simulink model "BCwithBPfix1"  (Simulink 7.0)
settings: Solver=FixedStepDiscrete  StartTime=0.0  StopTime=inf  FixedStep=0.001  RelTol=1e-3
libraries: dspsigops x84, dsPICdrivers x4
settings Model: Creator=Casparus  LastModifiedBy=Casparus  BufferReuse=off
settings OptimizationCC: BlockReduction=off  ConditionallyExecuteInputs=off  InlineParams=on  InlineInvariantSignals=on  OptimizeBlockIOStorage=off  BufferReuse=off  ExpressionFolding=off  LocalBlockOutputs=off  ZeroInternalMemoryAtStartup=off  InitFltsAndDblsToZero=off  EfficientFloat2IntCast=on  OptimizeModelRefInitCode=on
settings DebuggingCC: SignalInfNanChecking=error  ReadBeforeWriteMsg=EnableAllAsError  WriteAfterWriteMsg=EnableAllAsError  WriteAfterReadMsg=EnableAllAsError  AlgebraicLoopMsg=error  ArtificialAlgebraicLoopMsg=error  CheckExecutionContextPreStartOutputMsg=on  CheckExecutionContextRuntimeOutputMsg=on  BlockPriorityViolationMsg=error  SolverPrmCheckMsg=error  InheritedTsInSrcMsg=error  DiscreteInheritContinuousMsg=error  SigSpecEnsureSampleTimeMsg=error  CheckMatrixSingularityMsg=error  IntegerOverflowMsg=error  ParameterUnderflowMsg=error  ParameterPrecisionLossMsg=error  ParameterTunabilityLossMsg=error  UnderSpecifiedDataTypeMsg=error  UnnecessaryDatatypeConvMsg=warning  VectorMatrixConversionMsg=error  FcnCallInpInsideContextMsg=Enable All  SignalLabelMismatchMsg=error  UnconnectedInputMsg=error  UnconnectedOutputMsg=error  UnconnectedLineMsg=error  SFcnCompatibilityMsg=error  BusObjectLabelMismatch=error  RootOutportRequireBusObject=error  AssertControl=DisableAll  ModelReferenceIOMsg=error  ModelReferenceIOMismatchMessage=error  ModelReferenceCSMismatchMessage=warning  UnknownTsInhSupMsg=error  ModelReferenceDataLoggingMessage=error  StrictBusMsg=ErrorLevel1
settings HardwareCC: ProdBitPerInt=16  ProdEndianess=LittleEndian  ProdWordSize=16  ProdHWDeviceType=16-bit Generic
settings RTWCC: SystemTargetFile=dspic.tlc  TemplateMakefile=dspic_pic30_gcc.tmf  PostCodeGenCommand=dsPIC_Compile()  Description=Embedded Target for Microchip dsPIC (real-time)  ProcessScript=dspic_make_rtw_hook
settings CodeAppCC: ForceParamTrailComments=on  IgnoreCustomStorageClasses=off  MangleLength=4  ReqsInCode=on
settings STFCustomTargetCC: GenFloatMathFcnCalls=ANSI_C  ModelReferenceCompliant=off  IncludeMdlTerminateFcn=off  CombineOutputUpdateFcns=on  SuppressErrorStatus=on  ERTCustomFileBanners=on  SupportAbsoluteTime=off  SupportNonFinite=off  SupportContinuousTime=off  SupportNonInlinedSFcns=off  ParenthesesLevel=Maximum  SystemTargetFile=dspic.tlc
settings ERTTargetCC: GenFloatMathFcnCalls=ANSI_C  ModelReferenceCompliant=off  CompOptLevelCompliant=off  IncludeMdlTerminateFcn=off  SuppressErrorStatus=on  SupportAbsoluteTime=off  SupportNonFinite=off  ParenthesesLevel=Maximum  ModelStepFunctionPrototypeControlCompliant=off  ExtModeMexFile=noextcomm  InlinedParameterPlacement=NonHierarchical  ERTSrcFileBannerTemplate=dsPIC_code_template.cgt  ERTHdrFileBannerTemplate=dsPIC_code_template.cgt  ERTDataSrcFileTemplate=dsPIC_code_template.cgt  ERTDataHdrFileTemplate=dsPIC_code_template.cgt  ERTCustomFileTemplate=dsPIC_main.tlc  PreserveExpressionOrder=on  PreserveIfCondition=on
settings CustomProperty: DataType=string  Value=C:\PROGRA~1\MATLAB\R2007b\bin\win32\gmake

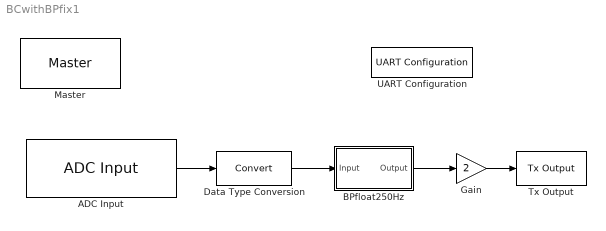
== system BCwithBPfix1 ==
  ADC Input : dsPICdrivers/Peripheral I//O/ADC Input  Tag=dsPIC_ADC  Priority=5  ADC_TYPE=12 bits  ADC_MODE=Continuous Sampling get output vector  NbrSampleStep=1  VoltRefpopup="External Vref+  -  AVss"  OutFormatBitspopup=0000 dddd dddd dddd : Integer  InterruptPriority=6  ANCHANNELS=[0]  MaxName=ANmax = 4096  Rin=1e2  ADCS=3  SAMC=1  Temperature=25  DMAChannel=0  SampleTime=0.001  Status="OK  |  Tsmp=8.000e-007 |  T/Channel=1.200e-005 |  Tall=1.200e-005"
  BPfloat250Hz : Subsystem  Tag=FilterWizardSubSystem
      settings: ErrorFcn=dspFilterRealizedInBasicElemsAlgLoopErrFcnCallback
  Data Type Conversion : DataTypeConversion  OutDataTypeMode=Specify via dialog
  Gain : Gain  Gain=2  ParameterDataType=sfix(16)  ParameterScaling=2^0  OutDataTypeMode=uint8  OutDataType=sfix(16)  OutScaling=2^0
  Master : dsPICdrivers/Master  Tag=dsPIC_MASTER  Priority=1  TimeStepType=Timer1  picType=30f4013  fcy=2.5e6  Quartz_33f=5e6  PLLActive_33f=off  fcyDesired_33f=0  tmr1="[1  2499  0]"  tmr1Info="Time Step : 0.001  ;   Error : 0%  PR1=2499"  tmr2345="[0  0  0  0]"  tmr2345cfg=[-1 -1 -1 -1]  IOautoConf=on  typePort="[ 0  0  0  0  0  0  0  0  0  0  0  0  0  0  0  0  8  0  0  0  0  0  0  0  0  0  0  0  0  0  0  0  0  0  0  0  0  0  0  0  0  0  0  0  0  0  0  0  0  0  0  0  0  0  0  0  0  0  0  0  0  0  0  0  0  0  0  0  0  0  0  0  0  0  0  0  0  0  0  0  0  0  4  5  0  0  0  0  0  0  0  0  0  0  0  0  0  0  0  0  0  0  0  0  0  0  0  0  0  0  0  0 ]"  TRIS="[ 65535  65535  65535  65535  65535  65535  65535 ]"  ADPCFG=0  MasterBusyPort=None  MasterOverloadPort=None  FOSC=XTL  TempProtection_33f=TEMP_ON  FPBOR=PBOR_OFF  PWRT=PWRT_OFF  MCLR=MCLR_DIS  PowerSave=off
  Tx Output : dsPICdrivers/Serial PORT/Tx Output  Tag=dsPIC_TX  Priority=5  UART=1  OrderingInOutPopup=None
  UART Configuration : dsPICdrivers/Serial PORT/UART Configuration  Tag=dsPIC_config_UART  Priority=2  UART=1  proposed_BAUD=9600  ALT_TX_RX=off  InterruptTxWhen=When Transmit Buffer is empty  TXInterruptPri=1  TxBufferSize=32  TXEN=on  InterruptRxWhen=When Receive Buffer is full (contain 4 characters)  RXInterruptPri=1  RxBufferSize=32  BAUD=9600  UxBRG=15  Info="UxBRG = 15   ||  Real Baud : 9766   ||  % error : 1.7253  ||  max 0.97656 Bytes / Step"  RealBaud=0
  wires:
  Gain/1 -> Tx Output/1
  ADC Input/1 -> Data Type Conversion/1
  Data Type Conversion/1 -> BPfloat250Hz/1(Input)
  BPfloat250Hz/1(Output) -> Gain/1

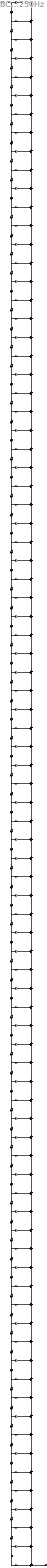
== system BCwithBPfix1/BPfloat250Hz ==
  Input : Inport
  BodyDelay{2..85} (84 alike) : dspsigops/Delay  Orientation=down  dly_unit=Samples  delay=1  ic_detail=off  dif_ic_for_ch=off  dif_ic_for_dly=off  ic=0  reset_popup=None
  BodyLSum{2..84} (83 alike) : Sum  Orientation=down  Inputs=++|  OutScaling=1  RndMeth=Nearest  SaturateOnIntegerOverflow=on
  BodyLSum85 : Sum  Inputs=++|  OutScaling=1  RndMeth=Nearest  SaturateOnIntegerOverflow=on
  b(1) : Gain  Gain=-0.00011400410035938231  ParameterDataTypeMode=Specify via dialog  ParameterDataType=float('double')  ParameterScalingMode=Use specified scaling  ParameterScaling=1  OutScaling=1  RndMeth=Nearest  SaturateOnIntegerOverflow=on
  b(10) : Gain  Gain=0.00076528749014445803  ParameterDataTypeMode=Specify via dialog  ParameterDataType=float('double')  ParameterScalingMode=Use specified scaling  ParameterScaling=1  OutScaling=1  RndMeth=Nearest  SaturateOnIntegerOverflow=on
  b(11) : Gain  Gain=-0.00055653560863696205  ParameterDataTypeMode=Specify via dialog  ParameterDataType=float('double')  ParameterScalingMode=Use specified scaling  ParameterScaling=1  OutScaling=1  RndMeth=Nearest  SaturateOnIntegerOverflow=on
  b(12) : Gain  Gain=-0.0017653960169033756  ParameterDataTypeMode=Specify via dialog  ParameterDataType=float('double')  ParameterScalingMode=Use specified scaling  ParameterScaling=1  OutScaling=1  RndMeth=Nearest  SaturateOnIntegerOverflow=on
  b(13) : Gain  Gain=0.00080126316068455581  ParameterDataTypeMode=Specify via dialog  ParameterDataType=float('double')  ParameterScalingMode=Use specified scaling  ParameterScaling=1  OutScaling=1  RndMeth=Nearest  SaturateOnIntegerOverflow=on
  b(14) : Gain  Gain=0.0033745175704345386  ParameterDataTypeMode=Specify via dialog  ParameterDataType=float('double')  ParameterScalingMode=Use specified scaling  ParameterScaling=1  OutScaling=1  RndMeth=Nearest  SaturateOnIntegerOverflow=on
  b(15) : Gain  Gain=-0.00084331270675375408  ParameterDataTypeMode=Specify via dialog  ParameterDataType=float('double')  ParameterScalingMode=Use specified scaling  ParameterScaling=1  OutScaling=1  RndMeth=Nearest  SaturateOnIntegerOverflow=on
  b(16) : Gain  Gain=-0.0057166316791322285  ParameterDataTypeMode=Specify via dialog  ParameterDataType=float('double')  ParameterScalingMode=Use specified scaling  ParameterScaling=1  OutScaling=1  RndMeth=Nearest  SaturateOnIntegerOverflow=on
  b(17) : Gain  Gain=0.0004479504040917559  ParameterDataTypeMode=Specify via dialog  ParameterDataType=float('double')  ParameterScalingMode=Use specified scaling  ParameterScaling=1  OutScaling=1  RndMeth=Nearest  SaturateOnIntegerOverflow=on
  b(18) : Gain  Gain=0.0088411131476842132  ParameterDataTypeMode=Specify via dialog  ParameterDataType=float('double')  ParameterScalingMode=Use specified scaling  ParameterScaling=1  OutScaling=1  RndMeth=Nearest  SaturateOnIntegerOverflow=on
  b(19) : Gain  Gain=0.00067442731314515544  ParameterDataTypeMode=Specify via dialog  ParameterDataType=float('double')  ParameterScalingMode=Use specified scaling  ParameterScaling=1  OutScaling=1  RndMeth=Nearest  SaturateOnIntegerOverflow=on
  b(2) : Gain  Gain=-0.00012559964702687091  ParameterDataTypeMode=Specify via dialog  ParameterDataType=float('double')  ParameterScalingMode=Use specified scaling  ParameterScaling=1  OutScaling=1  RndMeth=Nearest  SaturateOnIntegerOverflow=on
  b(20) : Gain  Gain=-0.012691969772935312  ParameterDataTypeMode=Specify via dialog  ParameterDataType=float('double')  ParameterScalingMode=Use specified scaling  ParameterScaling=1  OutScaling=1  RndMeth=Nearest  SaturateOnIntegerOverflow=on
  b(21) : Gain  Gain=-0.0028302241701637521  ParameterDataTypeMode=Specify via dialog  ParameterDataType=float('double')  ParameterScalingMode=Use specified scaling  ParameterScaling=1  OutScaling=1  RndMeth=Nearest  SaturateOnIntegerOverflow=on
  b(22) : Gain  Gain=0.017080765259904356  ParameterDataTypeMode=Specify via dialog  ParameterDataType=float('double')  ParameterScalingMode=Use specified scaling  ParameterScaling=1  OutScaling=1  RndMeth=Nearest  SaturateOnIntegerOverflow=on
  b(23) : Gain  Gain=0.0062943956875770521  ParameterDataTypeMode=Specify via dialog  ParameterDataType=float('double')  ParameterScalingMode=Use specified scaling  ParameterScaling=1  OutScaling=1  RndMeth=Nearest  SaturateOnIntegerOverflow=on
  b(24) : Gain  Gain=-0.021679640249729602  ParameterDataTypeMode=Specify via dialog  ParameterDataType=float('double')  ParameterScalingMode=Use specified scaling  ParameterScaling=1  OutScaling=1  RndMeth=Nearest  SaturateOnIntegerOverflow=on
  b(25) : Gain  Gain=-0.011251464760916772  ParameterDataTypeMode=Specify via dialog  ParameterDataType=float('double')  ParameterScalingMode=Use specified scaling  ParameterScaling=1  OutScaling=1  RndMeth=Nearest  SaturateOnIntegerOverflow=on
  b(26) : Gain  Gain=0.026040044883898328  ParameterDataTypeMode=Specify via dialog  ParameterDataType=float('double')  ParameterScalingMode=Use specified scaling  ParameterScaling=1  OutScaling=1  RndMeth=Nearest  SaturateOnIntegerOverflow=on
  b(27) : Gain  Gain=0.01774070618611993  ParameterDataTypeMode=Specify via dialog  ParameterDataType=float('double')  ParameterScalingMode=Use specified scaling  ParameterScaling=1  OutScaling=1  RndMeth=Nearest  SaturateOnIntegerOverflow=on
  b(28) : Gain  Gain=-0.029634639615999717  ParameterDataTypeMode=Specify via dialog  ParameterDataType=float('double')  ParameterScalingMode=Use specified scaling  ParameterScaling=1  OutScaling=1  RndMeth=Nearest  SaturateOnIntegerOverflow=on
  b(29) : Gain  Gain=-0.025613322377926483  ParameterDataTypeMode=Specify via dialog  ParameterDataType=float('double')  ParameterScalingMode=Use specified scaling  ParameterScaling=1  OutScaling=1  RndMeth=Nearest  SaturateOnIntegerOverflow=on
  b(3) : Gain  Gain=0.00014771328412910959  ParameterDataTypeMode=Specify via dialog  ParameterDataType=float('double')  ParameterScalingMode=Use specified scaling  ParameterScaling=1  OutScaling=1  RndMeth=Nearest  SaturateOnIntegerOverflow=on
  b(30) : Gain  Gain=0.031923272179050548  ParameterDataTypeMode=Specify via dialog  ParameterDataType=float('double')  ParameterScalingMode=Use specified scaling  ParameterScaling=1  OutScaling=1  RndMeth=Nearest  SaturateOnIntegerOverflow=on
  b(31) : Gain  Gain=0.034515179237363247  ParameterDataTypeMode=Specify via dialog  ParameterDataType=float('double')  ParameterScalingMode=Use specified scaling  ParameterScaling=1  OutScaling=1  RndMeth=Nearest  SaturateOnIntegerOverflow=on
  b(32) : Gain  Gain=-0.032431430566267301  ParameterDataTypeMode=Specify via dialog  ParameterDataType=float('double')  ParameterScalingMode=Use specified scaling  ParameterScaling=1  OutScaling=1  RndMeth=Nearest  SaturateOnIntegerOverflow=on
  b(33) : Gain  Gain=-0.043899732573517758  ParameterDataTypeMode=Specify via dialog  ParameterDataType=float('double')  ParameterScalingMode=Use specified scaling  ParameterScaling=1  OutScaling=1  RndMeth=Nearest  SaturateOnIntegerOverflow=on
  b(34) : Gain  Gain=0.030828713556614439  ParameterDataTypeMode=Specify via dialog  ParameterDataType=float('double')  ParameterScalingMode=Use specified scaling  ParameterScaling=1  OutScaling=1  RndMeth=Nearest  SaturateOnIntegerOverflow=on
  b(35) : Gain  Gain=0.053075176357706616  ParameterDataTypeMode=Specify via dialog  ParameterDataType=float('double')  ParameterScalingMode=Use specified scaling  ParameterScaling=1  OutScaling=1  RndMeth=Nearest  SaturateOnIntegerOverflow=on
  b(36) : Gain  Gain=-0.026994527169246309  ParameterDataTypeMode=Specify via dialog  ParameterDataType=float('double')  ParameterScalingMode=Use specified scaling  ParameterScaling=1  OutScaling=1  RndMeth=Nearest  SaturateOnIntegerOverflow=on
  b(37) : Gain  Gain=-0.061279551446267191  ParameterDataTypeMode=Specify via dialog  ParameterDataType=float('double')  ParameterScalingMode=Use specified scaling  ParameterScaling=1  OutScaling=1  RndMeth=Nearest  SaturateOnIntegerOverflow=on
  b(38) : Gain  Gain=0.021056309766186106  ParameterDataTypeMode=Specify via dialog  ParameterDataType=float('double')  ParameterScalingMode=Use specified scaling  ParameterScaling=1  OutScaling=1  RndMeth=Nearest  SaturateOnIntegerOverflow=on
  b(39) : Gain  Gain=0.067775120580984796  ParameterDataTypeMode=Specify via dialog  ParameterDataType=float('double')  ParameterScalingMode=Use specified scaling  ParameterScaling=1  OutScaling=1  RndMeth=Nearest  SaturateOnIntegerOverflow=on
  b(4) : Gain  Gain=5.5446602993773556e-005  ParameterDataTypeMode=Specify via dialog  ParameterDataType=float('double')  ParameterScalingMode=Use specified scaling  ParameterScaling=1  OutScaling=1  RndMeth=Nearest  SaturateOnIntegerOverflow=on
  b(40) : Gain  Gain=-0.013392258720000015  ParameterDataTypeMode=Specify via dialog  ParameterDataType=float('double')  ParameterScalingMode=Use specified scaling  ParameterScaling=1  OutScaling=1  RndMeth=Nearest  SaturateOnIntegerOverflow=on
  b(41) : Gain  Gain=-0.071946166637857939  ParameterDataTypeMode=Specify via dialog  ParameterDataType=float('double')  ParameterScalingMode=Use specified scaling  ParameterScaling=1  OutScaling=1  RndMeth=Nearest  SaturateOnIntegerOverflow=on
  b(42) : Gain  Gain=0.0045956094220973263  ParameterDataTypeMode=Specify via dialog  ParameterDataType=float('double')  ParameterScalingMode=Use specified scaling  ParameterScaling=1  OutScaling=1  RndMeth=Nearest  SaturateOnIntegerOverflow=on
  b(43) : Gain  Gain=0.073384080651335476  ParameterDataTypeMode=Specify via dialog  ParameterDataType=float('double')  ParameterScalingMode=Use specified scaling  ParameterScaling=1  OutScaling=1  RndMeth=Nearest  SaturateOnIntegerOverflow=on
  b(44) : Gain  Gain=0.0045956094220973263  ParameterDataTypeMode=Specify via dialog  ParameterDataType=float('double')  ParameterScalingMode=Use specified scaling  ParameterScaling=1  OutScaling=1  RndMeth=Nearest  SaturateOnIntegerOverflow=on
  b(45) : Gain  Gain=-0.071946166637857939  ParameterDataTypeMode=Specify via dialog  ParameterDataType=float('double')  ParameterScalingMode=Use specified scaling  ParameterScaling=1  OutScaling=1  RndMeth=Nearest  SaturateOnIntegerOverflow=on
  b(46) : Gain  Gain=-0.013392258720000015  ParameterDataTypeMode=Specify via dialog  ParameterDataType=float('double')  ParameterScalingMode=Use specified scaling  ParameterScaling=1  OutScaling=1  RndMeth=Nearest  SaturateOnIntegerOverflow=on
  b(47) : Gain  Gain=0.067775120580984796  ParameterDataTypeMode=Specify via dialog  ParameterDataType=float('double')  ParameterScalingMode=Use specified scaling  ParameterScaling=1  OutScaling=1  RndMeth=Nearest  SaturateOnIntegerOverflow=on
  b(48) : Gain  Gain=0.021056309766186106  ParameterDataTypeMode=Specify via dialog  ParameterDataType=float('double')  ParameterScalingMode=Use specified scaling  ParameterScaling=1  OutScaling=1  RndMeth=Nearest  SaturateOnIntegerOverflow=on
  b(49) : Gain  Gain=-0.061279551446267191  ParameterDataTypeMode=Specify via dialog  ParameterDataType=float('double')  ParameterScalingMode=Use specified scaling  ParameterScaling=1  OutScaling=1  RndMeth=Nearest  SaturateOnIntegerOverflow=on
  b(5) : Gain  Gain=-5.7332663760778328e-005  ParameterDataTypeMode=Specify via dialog  ParameterDataType=float('double')  ParameterScalingMode=Use specified scaling  ParameterScaling=1  OutScaling=1  RndMeth=Nearest  SaturateOnIntegerOverflow=on
  b(50) : Gain  Gain=-0.026994527169246309  ParameterDataTypeMode=Specify via dialog  ParameterDataType=float('double')  ParameterScalingMode=Use specified scaling  ParameterScaling=1  OutScaling=1  RndMeth=Nearest  SaturateOnIntegerOverflow=on
  b(51) : Gain  Gain=0.053075176357706616  ParameterDataTypeMode=Specify via dialog  ParameterDataType=float('double')  ParameterScalingMode=Use specified scaling  ParameterScaling=1  OutScaling=1  RndMeth=Nearest  SaturateOnIntegerOverflow=on
  b(52) : Gain  Gain=0.030828713556614439  ParameterDataTypeMode=Specify via dialog  ParameterDataType=float('double')  ParameterScalingMode=Use specified scaling  ParameterScaling=1  OutScaling=1  RndMeth=Nearest  SaturateOnIntegerOverflow=on
  b(53) : Gain  Gain=-0.043899732573517758  ParameterDataTypeMode=Specify via dialog  ParameterDataType=float('double')  ParameterScalingMode=Use specified scaling  ParameterScaling=1  OutScaling=1  RndMeth=Nearest  SaturateOnIntegerOverflow=on
  b(54) : Gain  Gain=-0.032431430566267301  ParameterDataTypeMode=Specify via dialog  ParameterDataType=float('double')  ParameterScalingMode=Use specified scaling  ParameterScaling=1  OutScaling=1  RndMeth=Nearest  SaturateOnIntegerOverflow=on
  b(55) : Gain  Gain=0.034515179237363247  ParameterDataTypeMode=Specify via dialog  ParameterDataType=float('double')  ParameterScalingMode=Use specified scaling  ParameterScaling=1  OutScaling=1  RndMeth=Nearest  SaturateOnIntegerOverflow=on
  b(56) : Gain  Gain=0.031923272179050548  ParameterDataTypeMode=Specify via dialog  ParameterDataType=float('double')  ParameterScalingMode=Use specified scaling  ParameterScaling=1  OutScaling=1  RndMeth=Nearest  SaturateOnIntegerOverflow=on
  b(57) : Gain  Gain=-0.025613322377926483  ParameterDataTypeMode=Specify via dialog  ParameterDataType=float('double')  ParameterScalingMode=Use specified scaling  ParameterScaling=1  OutScaling=1  RndMeth=Nearest  SaturateOnIntegerOverflow=on
  b(58) : Gain  Gain=-0.029634639615999717  ParameterDataTypeMode=Specify via dialog  ParameterDataType=float('double')  ParameterScalingMode=Use specified scaling  ParameterScaling=1  OutScaling=1  RndMeth=Nearest  SaturateOnIntegerOverflow=on
  b(59) : Gain  Gain=0.01774070618611993  ParameterDataTypeMode=Specify via dialog  ParameterDataType=float('double')  ParameterScalingMode=Use specified scaling  ParameterScaling=1  OutScaling=1  RndMeth=Nearest  SaturateOnIntegerOverflow=on
  b(6) : Gain  Gain=-2.1431167664734075e-005  ParameterDataTypeMode=Specify via dialog  ParameterDataType=float('double')  ParameterScalingMode=Use specified scaling  ParameterScaling=1  OutScaling=1  RndMeth=Nearest  SaturateOnIntegerOverflow=on
  b(60) : Gain  Gain=0.026040044883898328  ParameterDataTypeMode=Specify via dialog  ParameterDataType=float('double')  ParameterScalingMode=Use specified scaling  ParameterScaling=1  OutScaling=1  RndMeth=Nearest  SaturateOnIntegerOverflow=on
  b(61) : Gain  Gain=-0.011251464760916772  ParameterDataTypeMode=Specify via dialog  ParameterDataType=float('double')  ParameterScalingMode=Use specified scaling  ParameterScaling=1  OutScaling=1  RndMeth=Nearest  SaturateOnIntegerOverflow=on
  b(62) : Gain  Gain=-0.021679640249729602  ParameterDataTypeMode=Specify via dialog  ParameterDataType=float('double')  ParameterScalingMode=Use specified scaling  ParameterScaling=1  OutScaling=1  RndMeth=Nearest  SaturateOnIntegerOverflow=on
  b(63) : Gain  Gain=0.0062943956875770521  ParameterDataTypeMode=Specify via dialog  ParameterDataType=float('double')  ParameterScalingMode=Use specified scaling  ParameterScaling=1  OutScaling=1  RndMeth=Nearest  SaturateOnIntegerOverflow=on
  b(64) : Gain  Gain=0.017080765259904356  ParameterDataTypeMode=Specify via dialog  ParameterDataType=float('double')  ParameterScalingMode=Use specified scaling  ParameterScaling=1  OutScaling=1  RndMeth=Nearest  SaturateOnIntegerOverflow=on
  b(65) : Gain  Gain=-0.0028302241701637521  ParameterDataTypeMode=Specify via dialog  ParameterDataType=float('double')  ParameterScalingMode=Use specified scaling  ParameterScaling=1  OutScaling=1  RndMeth=Nearest  SaturateOnIntegerOverflow=on
  b(66) : Gain  Gain=-0.012691969772935312  ParameterDataTypeMode=Specify via dialog  ParameterDataType=float('double')  ParameterScalingMode=Use specified scaling  ParameterScaling=1  OutScaling=1  RndMeth=Nearest  SaturateOnIntegerOverflow=on
  b(67) : Gain  Gain=0.00067442731314515544  ParameterDataTypeMode=Specify via dialog  ParameterDataType=float('double')  ParameterScalingMode=Use specified scaling  ParameterScaling=1  OutScaling=1  RndMeth=Nearest  SaturateOnIntegerOverflow=on
  b(68) : Gain  Gain=0.0088411131476842132  ParameterDataTypeMode=Specify via dialog  ParameterDataType=float('double')  ParameterScalingMode=Use specified scaling  ParameterScaling=1  OutScaling=1  RndMeth=Nearest  SaturateOnIntegerOverflow=on
  b(69) : Gain  Gain=0.0004479504040917559  ParameterDataTypeMode=Specify via dialog  ParameterDataType=float('double')  ParameterScalingMode=Use specified scaling  ParameterScaling=1  OutScaling=1  RndMeth=Nearest  SaturateOnIntegerOverflow=on
  b(7) : Gain  Gain=-5.159828831138154e-005  ParameterDataTypeMode=Specify via dialog  ParameterDataType=float('double')  ParameterScalingMode=Use specified scaling  ParameterScaling=1  OutScaling=1  RndMeth=Nearest  SaturateOnIntegerOverflow=on
  b(70) : Gain  Gain=-0.0057166316791322285  ParameterDataTypeMode=Specify via dialog  ParameterDataType=float('double')  ParameterScalingMode=Use specified scaling  ParameterScaling=1  OutScaling=1  RndMeth=Nearest  SaturateOnIntegerOverflow=on
  b(71) : Gain  Gain=-0.00084331270675375408  ParameterDataTypeMode=Specify via dialog  ParameterDataType=float('double')  ParameterScalingMode=Use specified scaling  ParameterScaling=1  OutScaling=1  RndMeth=Nearest  SaturateOnIntegerOverflow=on
  b(72) : Gain  Gain=0.0033745175704345386  ParameterDataTypeMode=Specify via dialog  ParameterDataType=float('double')  ParameterScalingMode=Use specified scaling  ParameterScaling=1  OutScaling=1  RndMeth=Nearest  SaturateOnIntegerOverflow=on
  b(73) : Gain  Gain=0.00080126316068455581  ParameterDataTypeMode=Specify via dialog  ParameterDataType=float('double')  ParameterScalingMode=Use specified scaling  ParameterScaling=1  OutScaling=1  RndMeth=Nearest  SaturateOnIntegerOverflow=on
  b(74) : Gain  Gain=-0.0017653960169033756  ParameterDataTypeMode=Specify via dialog  ParameterDataType=float('double')  ParameterScalingMode=Use specified scaling  ParameterScaling=1  OutScaling=1  RndMeth=Nearest  SaturateOnIntegerOverflow=on
  b(75) : Gain  Gain=-0.00055653560863696205  ParameterDataTypeMode=Specify via dialog  ParameterDataType=float('double')  ParameterScalingMode=Use specified scaling  ParameterScaling=1  OutScaling=1  RndMeth=Nearest  SaturateOnIntegerOverflow=on
  b(76) : Gain  Gain=0.00076528749014445803  ParameterDataTypeMode=Specify via dialog  ParameterDataType=float('double')  ParameterScalingMode=Use specified scaling  ParameterScaling=1  OutScaling=1  RndMeth=Nearest  SaturateOnIntegerOverflow=on
  b(77) : Gain  Gain=0.00027927279700182126  ParameterDataTypeMode=Specify via dialog  ParameterDataType=float('double')  ParameterScalingMode=Use specified scaling  ParameterScaling=1  OutScaling=1  RndMeth=Nearest  SaturateOnIntegerOverflow=on
  b(78) : Gain  Gain=-0.00022768052715990187  ParameterDataTypeMode=Specify via dialog  ParameterDataType=float('double')  ParameterScalingMode=Use specified scaling  ParameterScaling=1  OutScaling=1  RndMeth=Nearest  SaturateOnIntegerOverflow=on
  b(79) : Gain  Gain=-5.159828831138154e-005  ParameterDataTypeMode=Specify via dialog  ParameterDataType=float('double')  ParameterScalingMode=Use specified scaling  ParameterScaling=1  OutScaling=1  RndMeth=Nearest  SaturateOnIntegerOverflow=on
  b(8) : Gain  Gain=-0.00022768052715990187  ParameterDataTypeMode=Specify via dialog  ParameterDataType=float('double')  ParameterScalingMode=Use specified scaling  ParameterScaling=1  OutScaling=1  RndMeth=Nearest  SaturateOnIntegerOverflow=on
  b(80) : Gain  Gain=-2.1431167664734075e-005  ParameterDataTypeMode=Specify via dialog  ParameterDataType=float('double')  ParameterScalingMode=Use specified scaling  ParameterScaling=1  OutScaling=1  RndMeth=Nearest  SaturateOnIntegerOverflow=on
  b(81) : Gain  Gain=-5.7332663760778328e-005  ParameterDataTypeMode=Specify via dialog  ParameterDataType=float('double')  ParameterScalingMode=Use specified scaling  ParameterScaling=1  OutScaling=1  RndMeth=Nearest  SaturateOnIntegerOverflow=on
  b(82) : Gain  Gain=5.5446602993773556e-005  ParameterDataTypeMode=Specify via dialog  ParameterDataType=float('double')  ParameterScalingMode=Use specified scaling  ParameterScaling=1  OutScaling=1  RndMeth=Nearest  SaturateOnIntegerOverflow=on
  b(83) : Gain  Gain=0.00014771328412910959  ParameterDataTypeMode=Specify via dialog  ParameterDataType=float('double')  ParameterScalingMode=Use specified scaling  ParameterScaling=1  OutScaling=1  RndMeth=Nearest  SaturateOnIntegerOverflow=on
  b(84) : Gain  Gain=-0.00012559964702687091  ParameterDataTypeMode=Specify via dialog  ParameterDataType=float('double')  ParameterScalingMode=Use specified scaling  ParameterScaling=1  OutScaling=1  RndMeth=Nearest  SaturateOnIntegerOverflow=on
  b(85) : Gain  Gain=-0.00011400410035938231  ParameterDataTypeMode=Specify via dialog  ParameterDataType=float('double')  ParameterScalingMode=Use specified scaling  ParameterScaling=1  OutScaling=1  RndMeth=Nearest  SaturateOnIntegerOverflow=on
  b(9) : Gain  Gain=0.00027927279700182126  ParameterDataTypeMode=Specify via dialog  ParameterDataType=float('double')  ParameterScalingMode=Use specified scaling  ParameterScaling=1  OutScaling=1  RndMeth=Nearest  SaturateOnIntegerOverflow=on
  Output : Outport
  wires:
  BodyLSum85/1 -> Output/1
  b(85)/1 -> BodyLSum85/2
  BodyDelay85/1 -> b(85)/1
  BodyLSum84/1 -> BodyLSum85/1
  b(84)/1 -> BodyLSum84/1
  BodyDelay84/1 -> BodyDelay85/1, b(84)/1
  BodyLSum83/1 -> BodyLSum84/2
  b(83)/1 -> BodyLSum83/1
  BodyDelay83/1 -> BodyDelay84/1, b(83)/1
  BodyLSum82/1 -> BodyLSum83/2
  b(82)/1 -> BodyLSum82/1
  BodyDelay82/1 -> BodyDelay83/1, b(82)/1
  BodyLSum81/1 -> BodyLSum82/2
  b(81)/1 -> BodyLSum81/1
  BodyDelay81/1 -> BodyDelay82/1, b(81)/1
  BodyLSum80/1 -> BodyLSum81/2
  b(80)/1 -> BodyLSum80/1
  BodyDelay80/1 -> BodyDelay81/1, b(80)/1
  BodyLSum79/1 -> BodyLSum80/2
  b(79)/1 -> BodyLSum79/1
  BodyDelay79/1 -> BodyDelay80/1, b(79)/1
  BodyLSum78/1 -> BodyLSum79/2
  b(78)/1 -> BodyLSum78/1
  BodyDelay78/1 -> BodyDelay79/1, b(78)/1
  BodyLSum77/1 -> BodyLSum78/2
  b(77)/1 -> BodyLSum77/1
  BodyDelay77/1 -> BodyDelay78/1, b(77)/1
  BodyLSum76/1 -> BodyLSum77/2
  b(76)/1 -> BodyLSum76/1
  BodyDelay76/1 -> BodyDelay77/1, b(76)/1
  BodyLSum75/1 -> BodyLSum76/2
  b(75)/1 -> BodyLSum75/1
  BodyDelay75/1 -> BodyDelay76/1, b(75)/1
  BodyLSum74/1 -> BodyLSum75/2
  b(74)/1 -> BodyLSum74/1
  BodyDelay74/1 -> BodyDelay75/1, b(74)/1
  BodyLSum73/1 -> BodyLSum74/2
  b(73)/1 -> BodyLSum73/1
  BodyDelay73/1 -> BodyDelay74/1, b(73)/1
  BodyLSum72/1 -> BodyLSum73/2
  b(72)/1 -> BodyLSum72/1
  BodyDelay72/1 -> BodyDelay73/1, b(72)/1
  BodyLSum71/1 -> BodyLSum72/2
  b(71)/1 -> BodyLSum71/1
  BodyDelay71/1 -> BodyDelay72/1, b(71)/1
  BodyLSum70/1 -> BodyLSum71/2
  b(70)/1 -> BodyLSum70/1
  BodyDelay70/1 -> BodyDelay71/1, b(70)/1
  BodyLSum69/1 -> BodyLSum70/2
  b(69)/1 -> BodyLSum69/1
  BodyDelay69/1 -> BodyDelay70/1, b(69)/1
  BodyLSum68/1 -> BodyLSum69/2
  b(68)/1 -> BodyLSum68/1
  BodyDelay68/1 -> BodyDelay69/1, b(68)/1
  BodyLSum67/1 -> BodyLSum68/2
  b(67)/1 -> BodyLSum67/1
  BodyDelay67/1 -> BodyDelay68/1, b(67)/1
  BodyLSum66/1 -> BodyLSum67/2
  b(66)/1 -> BodyLSum66/1
  BodyDelay66/1 -> BodyDelay67/1, b(66)/1
  BodyLSum65/1 -> BodyLSum66/2
  b(65)/1 -> BodyLSum65/1
  BodyDelay65/1 -> BodyDelay66/1, b(65)/1
  BodyLSum64/1 -> BodyLSum65/2
  b(64)/1 -> BodyLSum64/1
  BodyDelay64/1 -> BodyDelay65/1, b(64)/1
  BodyLSum63/1 -> BodyLSum64/2
  b(63)/1 -> BodyLSum63/1
  BodyDelay63/1 -> BodyDelay64/1, b(63)/1
  BodyLSum62/1 -> BodyLSum63/2
  b(62)/1 -> BodyLSum62/1
  BodyDelay62/1 -> BodyDelay63/1, b(62)/1
  BodyLSum61/1 -> BodyLSum62/2
  b(61)/1 -> BodyLSum61/1
  BodyDelay61/1 -> BodyDelay62/1, b(61)/1
  BodyLSum60/1 -> BodyLSum61/2
  b(60)/1 -> BodyLSum60/1
  BodyDelay60/1 -> BodyDelay61/1, b(60)/1
  BodyLSum59/1 -> BodyLSum60/2
  b(59)/1 -> BodyLSum59/1
  BodyDelay59/1 -> BodyDelay60/1, b(59)/1
  BodyLSum58/1 -> BodyLSum59/2
  b(58)/1 -> BodyLSum58/1
  BodyDelay58/1 -> BodyDelay59/1, b(58)/1
  BodyLSum57/1 -> BodyLSum58/2
  b(57)/1 -> BodyLSum57/1
  BodyDelay57/1 -> BodyDelay58/1, b(57)/1
  BodyLSum56/1 -> BodyLSum57/2
  b(56)/1 -> BodyLSum56/1
  BodyDelay56/1 -> BodyDelay57/1, b(56)/1
  BodyLSum55/1 -> BodyLSum56/2
  b(55)/1 -> BodyLSum55/1
  BodyDelay55/1 -> BodyDelay56/1, b(55)/1
  BodyLSum54/1 -> BodyLSum55/2
  b(54)/1 -> BodyLSum54/1
  BodyDelay54/1 -> BodyDelay55/1, b(54)/1
  BodyLSum53/1 -> BodyLSum54/2
  b(53)/1 -> BodyLSum53/1
  BodyDelay53/1 -> BodyDelay54/1, b(53)/1
  BodyLSum52/1 -> BodyLSum53/2
  b(52)/1 -> BodyLSum52/1
  BodyDelay52/1 -> BodyDelay53/1, b(52)/1
  BodyLSum51/1 -> BodyLSum52/2
  b(51)/1 -> BodyLSum51/1
  BodyDelay51/1 -> BodyDelay52/1, b(51)/1
  BodyLSum50/1 -> BodyLSum51/2
  b(50)/1 -> BodyLSum50/1
  BodyDelay50/1 -> BodyDelay51/1, b(50)/1
  BodyLSum49/1 -> BodyLSum50/2
  b(49)/1 -> BodyLSum49/1
  BodyDelay49/1 -> BodyDelay50/1, b(49)/1
  BodyLSum48/1 -> BodyLSum49/2
  b(48)/1 -> BodyLSum48/1
  BodyDelay48/1 -> BodyDelay49/1, b(48)/1
  BodyLSum47/1 -> BodyLSum48/2
  b(47)/1 -> BodyLSum47/1
  BodyDelay47/1 -> BodyDelay48/1, b(47)/1
  BodyLSum46/1 -> BodyLSum47/2
  b(46)/1 -> BodyLSum46/1
  BodyDelay46/1 -> BodyDelay47/1, b(46)/1
  BodyLSum45/1 -> BodyLSum46/2
  b(45)/1 -> BodyLSum45/1
  BodyDelay45/1 -> BodyDelay46/1, b(45)/1
  BodyLSum44/1 -> BodyLSum45/2
  b(44)/1 -> BodyLSum44/1
  BodyDelay44/1 -> BodyDelay45/1, b(44)/1
  BodyLSum43/1 -> BodyLSum44/2
  b(43)/1 -> BodyLSum43/1
  BodyDelay43/1 -> BodyDelay44/1, b(43)/1
  BodyLSum42/1 -> BodyLSum43/2
  b(42)/1 -> BodyLSum42/1
  BodyDelay42/1 -> BodyDelay43/1, b(42)/1
  BodyLSum41/1 -> BodyLSum42/2
  b(41)/1 -> BodyLSum41/1
  BodyDelay41/1 -> BodyDelay42/1, b(41)/1
  BodyLSum40/1 -> BodyLSum41/2
  b(40)/1 -> BodyLSum40/1
  BodyDelay40/1 -> BodyDelay41/1, b(40)/1
  BodyLSum39/1 -> BodyLSum40/2
  b(39)/1 -> BodyLSum39/1
  BodyDelay39/1 -> BodyDelay40/1, b(39)/1
  BodyLSum38/1 -> BodyLSum39/2
  b(38)/1 -> BodyLSum38/1
  BodyDelay38/1 -> BodyDelay39/1, b(38)/1
  BodyLSum37/1 -> BodyLSum38/2
  b(37)/1 -> BodyLSum37/1
  BodyDelay37/1 -> BodyDelay38/1, b(37)/1
  BodyLSum36/1 -> BodyLSum37/2
  b(36)/1 -> BodyLSum36/1
  BodyDelay36/1 -> BodyDelay37/1, b(36)/1
  BodyLSum35/1 -> BodyLSum36/2
  b(35)/1 -> BodyLSum35/1
  BodyDelay35/1 -> BodyDelay36/1, b(35)/1
  BodyLSum34/1 -> BodyLSum35/2
  b(34)/1 -> BodyLSum34/1
  BodyDelay34/1 -> BodyDelay35/1, b(34)/1
  BodyLSum33/1 -> BodyLSum34/2
  b(33)/1 -> BodyLSum33/1
  BodyDelay33/1 -> BodyDelay34/1, b(33)/1
  BodyLSum32/1 -> BodyLSum33/2
  b(32)/1 -> BodyLSum32/1
  BodyDelay32/1 -> BodyDelay33/1, b(32)/1
  BodyLSum31/1 -> BodyLSum32/2
  b(31)/1 -> BodyLSum31/1
  BodyDelay31/1 -> BodyDelay32/1, b(31)/1
  BodyLSum30/1 -> BodyLSum31/2
  b(30)/1 -> BodyLSum30/1
  BodyDelay30/1 -> BodyDelay31/1, b(30)/1
  BodyLSum29/1 -> BodyLSum30/2
  b(29)/1 -> BodyLSum29/1
  BodyDelay29/1 -> BodyDelay30/1, b(29)/1
  BodyLSum28/1 -> BodyLSum29/2
  b(28)/1 -> BodyLSum28/1
  BodyDelay28/1 -> BodyDelay29/1, b(28)/1
  BodyLSum27/1 -> BodyLSum28/2
  b(27)/1 -> BodyLSum27/1
  BodyDelay27/1 -> BodyDelay28/1, b(27)/1
  BodyLSum26/1 -> BodyLSum27/2
  b(26)/1 -> BodyLSum26/1
  BodyDelay26/1 -> BodyDelay27/1, b(26)/1
  BodyLSum25/1 -> BodyLSum26/2
  b(25)/1 -> BodyLSum25/1
  BodyDelay25/1 -> BodyDelay26/1, b(25)/1
  BodyLSum24/1 -> BodyLSum25/2
  b(24)/1 -> BodyLSum24/1
  BodyDelay24/1 -> BodyDelay25/1, b(24)/1
  BodyLSum23/1 -> BodyLSum24/2
  b(23)/1 -> BodyLSum23/1
  BodyDelay23/1 -> BodyDelay24/1, b(23)/1
  BodyLSum22/1 -> BodyLSum23/2
  b(22)/1 -> BodyLSum22/1
  BodyDelay22/1 -> BodyDelay23/1, b(22)/1
  BodyLSum21/1 -> BodyLSum22/2
  b(21)/1 -> BodyLSum21/1
  BodyDelay21/1 -> BodyDelay22/1, b(21)/1
  BodyLSum20/1 -> BodyLSum21/2
  b(20)/1 -> BodyLSum20/1
  BodyDelay20/1 -> BodyDelay21/1, b(20)/1
  BodyLSum19/1 -> BodyLSum20/2
  b(19)/1 -> BodyLSum19/1
  BodyDelay19/1 -> BodyDelay20/1, b(19)/1
  BodyLSum18/1 -> BodyLSum19/2
  b(18)/1 -> BodyLSum18/1
  BodyDelay18/1 -> BodyDelay19/1, b(18)/1
  BodyLSum17/1 -> BodyLSum18/2
  b(17)/1 -> BodyLSum17/1
  BodyDelay17/1 -> BodyDelay18/1, b(17)/1
  BodyLSum16/1 -> BodyLSum17/2
  b(16)/1 -> BodyLSum16/1
  BodyDelay16/1 -> BodyDelay17/1, b(16)/1
  BodyLSum15/1 -> BodyLSum16/2
  b(15)/1 -> BodyLSum15/1
  BodyDelay15/1 -> BodyDelay16/1, b(15)/1
  BodyLSum14/1 -> BodyLSum15/2
  b(14)/1 -> BodyLSum14/1
  BodyDelay14/1 -> BodyDelay15/1, b(14)/1
  BodyLSum13/1 -> BodyLSum14/2
  b(13)/1 -> BodyLSum13/1
  BodyDelay13/1 -> BodyDelay14/1, b(13)/1
  BodyLSum12/1 -> BodyLSum13/2
  b(12)/1 -> BodyLSum12/1
  BodyDelay12/1 -> BodyDelay13/1, b(12)/1
  BodyLSum11/1 -> BodyLSum12/2
  b(11)/1 -> BodyLSum11/1
  BodyDelay11/1 -> BodyDelay12/1, b(11)/1
  BodyLSum10/1 -> BodyLSum11/2
  b(10)/1 -> BodyLSum10/1
  BodyDelay10/1 -> BodyDelay11/1, b(10)/1
  BodyLSum9/1 -> BodyLSum10/2
  b(9)/1 -> BodyLSum9/1
  BodyDelay9/1 -> BodyDelay10/1, b(9)/1
  BodyLSum8/1 -> BodyLSum9/2
  b(8)/1 -> BodyLSum8/1
  BodyDelay8/1 -> BodyDelay9/1, b(8)/1
  BodyLSum7/1 -> BodyLSum8/2
  b(7)/1 -> BodyLSum7/1
  BodyDelay7/1 -> BodyDelay8/1, b(7)/1
  BodyLSum6/1 -> BodyLSum7/2
  b(6)/1 -> BodyLSum6/1
  BodyDelay6/1 -> BodyDelay7/1, b(6)/1
  BodyLSum5/1 -> BodyLSum6/2
  b(5)/1 -> BodyLSum5/1
  BodyDelay5/1 -> BodyDelay6/1, b(5)/1
  BodyLSum4/1 -> BodyLSum5/2
  b(4)/1 -> BodyLSum4/1
  BodyDelay4/1 -> BodyDelay5/1, b(4)/1
  BodyLSum3/1 -> BodyLSum4/2
  b(3)/1 -> BodyLSum3/1
  BodyDelay3/1 -> BodyDelay4/1, b(3)/1
  BodyLSum2/1 -> BodyLSum3/2
  b(2)/1 -> BodyLSum2/1
  BodyDelay2/1 -> BodyDelay3/1, b(2)/1
  b(1)/1 -> BodyLSum2/2
  Input/1 -> BodyDelay2/1, b(1)/1
